simulink model "Off-Board-EV-Charger"  (R2018a)
settings: Solver=ode23tb  StartTime=0.0  StopTime=4  FixedStep=2.5e-6  MaxStep=1e-5  RelTol=1e-3  AbsTol=1e-5
undefined symbols (not defined in the file): Ion, Lithium
libraries: powerlib x22, simulink x7, powerlib_meascontrol x5, powerlib_extras x2, electricdrivelib x1, re_lib x1
settings Model: Creator=hp  LastModifiedBy=ADMIN
settings SolverCC: ZeroCrossControl=DisableAll  ZeroCrossAlgorithm=Adaptive  AlgebraicLoopSolver=LineSearch
settings DataIOCC: ReturnWorkspaceOutputs=on  Refine=2
settings DebuggingCC: AlgebraicLoopMsg=none  MaskedZcDiagnostic=none  IgnoredZcDiagnostic=none  UnconnectedInputMsg=none  UnconnectedOutputMsg=none  UnconnectedLineMsg=none
settings ModelReferenceCC: EnableRefExpFcnMdlSchedulingChecks=off
settings SFSimCC: SimUseLocalCustomCode=on
settings RTWCC: Description=Generic Real-Time Target  RTWUseLocalCustomCode=on

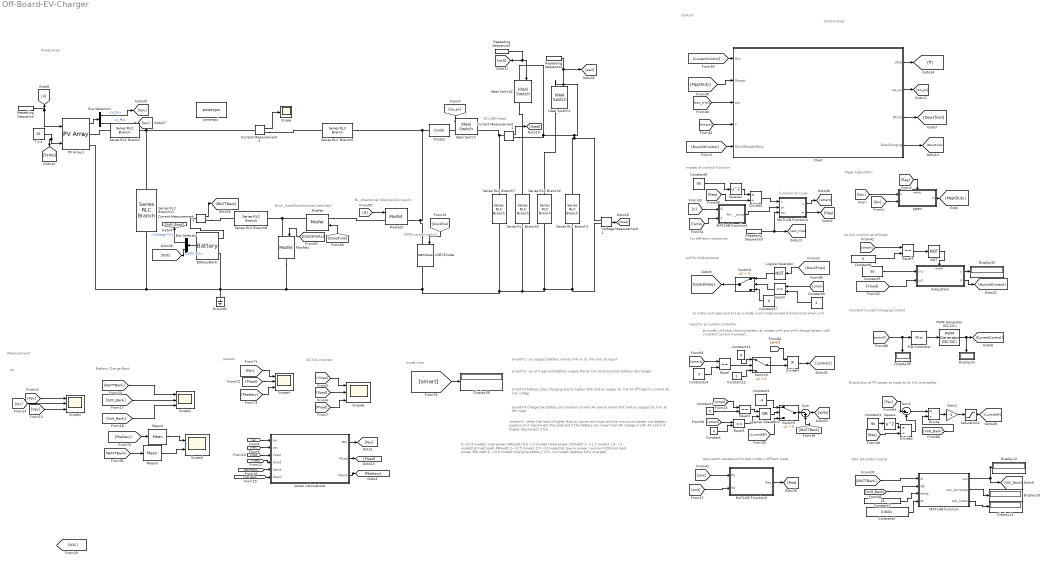
== system Off-Board-EV-Charger ==
  note: Buck_boost(bidrectional switches)
  note: DCLINK+load
  note: BI _directional (block/allow)
      | swich
  note: MPPt control switch
  note: mode view
  note: 0-->0.5 mode1( load power  306watt)
      | 0.5-->1 mode4 (load power  253watt)
      | 1-->1.5 mode3
      | 1.5-->2 mode2(at high load) 490watt
      | 2-->2.5 mode1
      | 2.5-->3 mode2(at low pv power ) pvmax=200 and load power 306 watt
      | 3-->3.5 mode5 (charging battery)
      | 3.5-->4 mode5 (battery fully charged
  note: dc link controll at offmppt
  note: Mppt Alghorithm
  note: Constant Current Charging Control
  note: powers
  note: DC link monitor
  note: Battery Charge Bank
  note: PV
  note: Measurement
  note: Control
  note: Power Area
  note: Distrbution of PV power at mppt to dc link and battey
  note: Control Area
  note: smart=1 : pv supplys battery and dc link or dc link only at mpp t
  note: smart=4 charge the battery at constant current 4A due to lower SOC and pv supplys dc link at off mppt
  note: smart=3 battery stop charging due to higher SOC and pv supply dc link at offmppt to control dc link voltge
  note: smart=5 : when the load is higher than pv power at mmpt and the maximum power can battery supplys so it disconnect the load and if the battery soc lower than 90 charge it with 4A and if it higher disconnect it too
  note: smart=2 : pv at mppt and battery supply the dc link (bidirectional battery discharge)
  note: function of mods
  note: for diffrent Irradiances
  note: modes of controll function
  note: sw3 for bidirectional
  note: to make sw3 open and act as a diode in all mods except bidirectional when y=2
  note: input for pi current controller
  note: at mode y=3 stop charing battery at modes y=5 and y=4 charge battery with constant current 4 ampers
  note: equivalent resistance for test mods in diffrent loads
  note: SOC Estimatorl trailer
  BatteryBank : electricdrivelib/Extra Sources/Battery  BatType=Lithium-Ion  ShowTempParam=off  ThermalPreset=no  ShowAgeParam=off  NomV=21.8  NomQ=12  SOC=80  Batt_Tr=1  PresetModel=on  MaxQ=12  MinV=16.35  FullV=25.3749  Dis_rate=5.2174  R=0.018167  Normal_OP=10.8522  expZone="[23.5524     0.589565]"  current=[6.5 13 32.5]  Units=Time  Tci=20  NomT=20  T2=-30  MaxQ2=4.8  FullV2=7.1  Normal_OP2=5.655  expZone2="[6.58           1]"  Rca=0.6  ti=2000  Dp=0  Neq0=0  Tsim=1e6  Ta1=25  Qeol=5.4*0.9  Reol=0.013333*1.2  Char_age=[2.3478, 3]  Dis_age=[2.3478, 10]  N1=1500  N2=10500  N3=1000  N4=1400  Ta2=45  N5=950
  Bus Selector : BusSelector  OutputSignals=Voltage (V),SOC (%)
  Bus Selector1 : BusSelector  OutputSignals=V_PV,I_PV
  Chart : Stateflow chart  TreatAsAtomicUnit=on
  Constant : Constant  Value=4
  Constant1 : Constant  Value=90
  Constant11 : Constant  Value=0
  Constant12 : Constant
  Constant17 : Constant  Value=0
  Constant2 : Constant  Value=0.0001
  Constant24 : Constant  Value=3
  Constant3 : Constant  Value=5
  Constant4 : Constant  Value=-4
  Constant5 : Constant  Value=90
  Constant6 : Constant  Value=5
  Constant7 : Constant  Value=25
  Constant8 : Constant  Value=2
  Constant9 : Constant  Value=90
  Current Measurement1 : powerlib/Measurements/Current Measurement  PhasorSimulation=off  OutputType=Complex  PSBequivalent=0
  Current Measurement2 : powerlib/Measurements/Current Measurement  PhasorSimulation=off  OutputType=Complex  PSBequivalent=0
  Current Measurement3 : powerlib/Measurements/Current Measurement  PhasorSimulation=off  OutputType=Complex  PSBequivalent=0
  Diode1 : powerlib/Power Electronics/Diode  Ron=0.001  Lon=0  Vf=0.8  IC=0  UseSnubber=0  Rs=500  Cs=250e-9  Measurements=off
  Display{10..12,30..31,33,38} (7 alike) : Display
  Divide : Product  Inputs=*/
  Divide2 : Product  Inputs=*/
  Divide4 : Product  Inputs=**
  Divide5 : Product  Inputs=*/
  Equal{,1..4} (5 alike) : RelationalOperator  Operator===  OutDataTypeStr=boolean  RndMeth=Simplest
  Gain1 : Gain  Gain=-1
  Ground2 : powerlib/Elements/Ground  LConnTagsString=a
  IGBT/Diode : powerlib/Power Electronics/IGBT//Diode  Ron=1e-3  Rs=1e5  Cs=inf  Measurements=on
  Ideal Switch : powerlib/Power Electronics/Ideal Switch  Ron=0.001  Lon=0  IC=0  Rs=1e5  Cs=inf  Measurements=on
  Ideal Switch1 : powerlib/Power Electronics/Ideal Switch  Ron=0.001  Lon=0  IC=0  Rs=1e5  Cs=inf  Measurements=on
  Ideal Switch2 : powerlib/Power Electronics/Ideal Switch  Ron=0.001  Lon=0  IC=0  Rs=1e5  Cs=inf  Measurements=on
  Logical Operator : Logic  Operator=NOT  AllPortsSameDT=off  OutDataTypeStr=boolean
  Logical Operator1 : Logic  Operator=OR  AllPortsSameDT=off  OutDataTypeStr=boolean
  MATLAB Function : MATLAB Function  TreatAsAtomicUnit=on
  MATLAB Function1 : MATLAB Function  TreatAsAtomicUnit=on
  MATLAB Function2 : MATLAB Function  TreatAsAtomicUnit=on
  MATLAB Function3 : MATLAB Function  TreatAsAtomicUnit=on
  MPPT : Subsystem
  Mean3 : powerlib_meascontrol/Measurements/Mean  Freq=50  Vinit=0  Ts=0
  Mean4 : powerlib_meascontrol/Measurements/Mean  Freq=50  Vinit=0  Ts=0
  Mosfet : powerlib/Power Electronics/Mosfet  Ron=0.1  Lon=0  Rd=0.01  Vfd=0  IC=0  Rs=1e5  Cs=inf  Measurements=on
  Mosfet1 : powerlib/Power Electronics/Mosfet  Ron=0.1  Lon=0  Rd=0.01  Vfd=0  IC=0  Rs=1e5  Cs=inf  Measurements=off
  Mosfet2 : powerlib/Power Electronics/Mosfet  Ron=0.1  Lon=0  Rd=0.01  Vfd=0  IC=0  Rs=1e5  Cs=inf  Measurements=on
  NOT : Logic  Operator=NOT  IconShape=distinctive  AllPortsSameDT=off  OutDataTypeStr=boolean
  PID Controller : simulink/Continuous/PID Controller  Controller=PI  TimeDomain=Continuous-time  SampleTime=-1  IntegratorMethod=Forward Euler  FilterMethod=Forward Euler  Form=Parallel  UseFilter=on  ControllerParametersSource=internal  P=25  I=5000  D=0  N=100  InitialConditionSource=internal  InitialConditionForIntegrator=0  InitialConditionForFilter=0  ExternalReset=none  LimitOutput=on  UpperSaturationLimit=0.95  LowerSaturationLimit=0  LinearizeAsGain=on  AntiWindupMode=clamping  Kb=1  TrackingMode=off  Kt=1  PParamMin=[]  PParamMax=[]  IParamMin=[]  IParamMax=[]  DParamMin=[]  DParamMax=[]  NParamMin=[]  NParamMax=[]  KbParamMin=[]  KbParamMax=[]  KtParamMin=[]  KtParamMax=[]  POutMin=[]  POutMax=[]  IOutMin=[]  IOutMax=[]  DOutMin=[]  DOutMax=[]  NOutMin=[]  NOutMax=[]  KbOutMin=[]  KbOutMax=[]  KtOutMin=[]  KtOutMax=[]  IntegratorOutMin=[]  IntegratorOutMax=[]  FilterOutMin=[]  FilterOutMax=[]  SumOutMin=[]  SumOutMax=[]  SumI1OutMin=[]  SumI1OutMax=[]  SumI2OutMin=[]  SumI2OutMax=[]  SumI3OutMin=[]  SumI3OutMax=[]  SumDOutMin=[]  SumDOutMax=[]  SaturationOutMin=[]  SaturationOutMax=[]  IntegratorContinuousStateAttributes=''  IntegratorStateMustResolveToSignalObject=off  IntegratorRTWStateStorageClass=Auto  FilterContinuousStateAttributes=''  FilterStateMustResolveToSignalObject=off  FilterRTWStateStorageClass=Auto  DifferentiatorICPrevScaledInput=0  DifferentiatorOutMin=[]  DifferentiatorOutMax=[]  FilterDiffOutCoefMin=[]  FilterDiffOutCoefMax=[]  SumDenOutMin=[]  SumDenOutMax=[]  SumNumOutMin=[]  SumNumOutMax=[]  ReciprocalOutMin=[]  ReciprocalOutMax=[]  DivideOutMin=[]  DivideOutMax=[]  TunerSelectOption=Transfer Function Based (PID Tuner App)
  PV Array1 : re_lib/Solar/PV Array  Npar=1  Nser=4  PlotType=array @ 25 deg.C & specified irradiances  S_vec="[ 1000   ]"  Temp_C_vec="[ 45 25  ]"  ModuleName=User-defined  PlotWhenSelected=off  Pm=99.925  Ncell=60  Voc=21.9  Isc=6.09  Vm=17.5  Im=5.71  beta_Voc_pc=-0.36099  alpha_Isc_pc=0.102  beta_Voc=-0.079057  alpha_Isc=0.0062118  IL=6.1019  I0=2.2502e-10  nI=0.59168  Rsh=284.8348  Rs=0.30531  BAL=off  Tc=1e-6  Tfilter=5e-5
  PWM Generator (DC-DC) : powerlib_meascontrol/Pulse & Signal Generators/PWM Generator (DC-DC)  Fsw=20000  Ts=0
  Repeating Sequence : simulink/Sources/Repeating Sequence  rep_seq_t="[0 2.5 2.5+1e-9 3  3.00000001 3.5 4]"  rep_seq_y="[1000 1000  500 500 250 250 250]"
  Repeating Sequence1 : simulink/Sources/Repeating Sequence  rep_seq_t=[0 0.5 0.5+1e-9 1.5 1.5+1e-9 4]  rep_seq_y=[1 1 0 0 1 1]
  Repeating Sequence2 : simulink/Sources/Repeating Sequence  rep_seq_t=[0 0.5 0.5+1e-9 1.5 1.5+1e-9 2 2.0000001 3.5 4]  rep_seq_y=[0 0 0 0 1 1 0 0 0]
  Repeating Sequence3 : simulink/Sources/Repeating Sequence  rep_seq_t=[0 0.5 1 1.5 2 2.5 3 3.5 4]  rep_seq_y=[10 50 90 90 50 70 10 90 90]
  Saturation2 : Saturate  UpperLimit=5  LowerLimit=-5
  Scope : Scope
  Scope{1..2,4,6} (4 alike) : Scope  NumInputPorts=3
  Scope3 : Scope  NumInputPorts=2
  Series RLC Branch : powerlib/Elements/Series RLC Branch  LConnTagsString=__new0  RConnTagsString=__new0  BranchType=R  Resistance=0.1  Inductance=1e-3  SetiL0=off  InitialCurrent=0  Capacitance=1e-6  Setx0=off  InitialVoltage=0  Measurements=None
  Series RLC Branch1 : powerlib/Elements/Series RLC Branch  LConnTagsString=__new0  RConnTagsString=__new0  BranchType=R  Resistance=32  Inductance=1e-3  SetiL0=off  InitialCurrent=0  Capacitance=0.0134  Setx0=off  InitialVoltage=50  Measurements=None
  Series RLC Branch11 : powerlib/Elements/Series RLC Branch  LConnTagsString=__new0  RConnTagsString=__new0  BranchType=C  Resistance=0.1  Inductance=1e-3  SetiL0=off  InitialCurrent=0  Capacitance=1000e-6  Setx0=off  InitialVoltage=0  Measurements=None
  Series RLC Branch2 : powerlib/Elements/Series RLC Branch  LConnTagsString=__new0  RConnTagsString=__new0  BranchType=R  Resistance=152.5  Inductance=1e-3  SetiL0=off  InitialCurrent=0  Capacitance=0.0134  Setx0=off  InitialVoltage=50  Measurements=None
  Series RLC Branch3 : powerlib/Elements/Series RLC Branch  LConnTagsString=__new0  RConnTagsString=__new0  BranchType=R  Resistance=43.86  Inductance=1e-3  SetiL0=off  InitialCurrent=0  Capacitance=0.0134  Setx0=off  InitialVoltage=50  Measurements=None
  Series RLC Branch6 : powerlib/Elements/Series RLC Branch  LConnTagsString=__new0  RConnTagsString=__new0  BranchType=L  Resistance=1  Inductance=13.5e-3  SetiL0=off  InitialCurrent=55  Capacitance=1e-6  Setx0=off  InitialVoltage=0  Measurements=None
  Series RLC Branch7 : powerlib/Elements/Series RLC Branch  LConnTagsString=__new0  RConnTagsString=__new0  BranchType=C  Resistance=0.0016  Inductance=1e-3  SetiL0=off  InitialCurrent=0  Capacitance=1000e-6  Setx0=off  InitialVoltage=50  Measurements=None
  Series RLC Branch8 : powerlib/Elements/Series RLC Branch  LConnTagsString=__new0  RConnTagsString=__new0  BranchType=L  Resistance=1  Inductance=3.5e-3  SetiL0=off  InitialCurrent=4  Capacitance=1e-6  Setx0=off  InitialVoltage=0  Measurements=None
  Square : Math  Operator=square  SaturateOnIntegerOverflow=on
  Square1 : Math  Operator=square  SaturateOnIntegerOverflow=on
  Subsystem : Subsystem
  Sum : Sum  Inputs=|-+
  Sum1 : Sum  Inputs=|+-
  Switch3 : Switch  Criteria=u2 > Threshold
  Switch4 : Switch  Criteria=u2 > Threshold
  Switch5 : Switch  Criteria=u2 > Threshold
  T in1 : Constant  Value=25
  Voltage Measurement1 : powerlib/Measurements/Voltage Measurement  PhasorSimulation=off  OutputType=Complex  PSBequivalent=0
  "power calculations " : Subsystem
  powergui : powerlib/powergui  Priority=1  SimulationMode=Discrete  SampleTime=5e-6  frequency=60  Iterations=50  frequencyindice=0  Pbase=100e6  ErrMax=1e-4  UnitsV=kV  UnitsW=MW  buscounter=0  FunctionMessages=off  echomessages=off  EnableUseOfTLC=off  CurrentSourceSwitches=off  DisableSnubberDevices=off  DisableRonSwitches=off  DisableVfSwitches=off  DisplayEquations=off  SolverType=Tustin/Backward Euler (TBE)  Interpol=off  ExternalGateDelay=off  methode=off  Ts=100  x0status=blocks  SPID=on  SwTol=0  HookPort=off  RestoreLinks=warning  ResistiveCurrentMeasurement=off  Frange=[0:2:500]  Ylog=off  Xlog=on  ShowGrid=off  save=off  variable=ZData  structure=0  ZoomFFT=off  StartTime=0.0  cycles=1  DisplayStyle=1  fundamental=60  FreqAxis=off  MaxFrequency=1000  frequencyindicesteady=1  RmsSteady=1  display=off
  wires:
  Current Measurement1/1 -> [Iload]
  T in1/1 -> PV Array1/2, [Temp]
  Bus Selector1/2 -> [Ipv]  "<I_PV>"
  Bus Selector1/1 -> [Vpv]  "<V_PV>"
  PV Array1/1 -> Bus Selector1/1
  Current Measurement3/1 -> [IBATTBank]
  BatteryBank/1 -> Bus Selector/1
  [Vload] -> Scope6/1
  [Iload] -> Scope6/2
  [Pload] -> Scope6/3
  [Ppv] -> Scope2/1
  Bus Selector/1 -> [Volt_Bank]  "<Voltage (V)>"
  [IBATTBank] -> Scope1/1
  [Volt_Bank] -> Scope1/3
  [SOC_Bank] -> Scope1/2
  PWM Generator (DC-DC)/1 -> [CurrentControl], Display31/1
  PID Controller/1 -> PWM Generator (DC-DC)/1
  [Ipv] -> MPPT/2(I)
  [Vpv] -> MPPT/1(V)
  Voltage Measurement1/1 -> [Vload]
  Divide/1 -> Gain1/1
  Sum1/1 -> Divide/1
  [Volt_Bank] -> Divide/2
  Bus Selector/2 -> [SOC]  "<SOC (%)>"
  [IBATTBank] -> Mean3/1
  Mean3/1 -> Scope3/2
  [BusVoltControl] -> Chart/5(DcLinkSupplyDuty)
  [CurrentControl] -> Chart/1(Dcc)
  Chart/3(Dfinal) -> [Dsw1final]
  Chart/4(DutyCharging) -> [Dsw2Final]
  Constant1/1 -> Square/1
  Square/1 -> Divide2/1
  Divide2/1 -> Sum1/2
  [control2] -> Display30/1, PID Controller/1
  [Dsw2Final] -> Mosfet/1
  Gain1/1 -> Saturation2/1
  Saturation2/1 -> [CurrentREF]
  [ff] -> Mosfet2/1
  [smart] -> Chart/4(Y)
  [DSW3FINAL] -> Mosfet1/1
  [MpptDuty] -> Chart/2(Dmppt)
  [Req] -> Divide2/2
  [Ppv] -> Sum1/1
  Chart/1(data) -> [ff]
  [Pbattery] -> Scope4/3
  [Ppv] -> Scope4/1
  [Pload] -> Scope4/2
  [smart] -> Display38/1
  MPPT/1(D) -> [MpptDuty]
  [flag] -> MPPT/Enable
  Chart/2(sw_pv) -> [sw_pv]
  [Dsw1final] -> IGBT/Diode/1
  [sw_pv] -> Ideal Switch/1
  [soc_trial] -> Chart/3(soc)
  Constant5/1 -> Subsystem/1(In1)
  [Vload] -> Subsystem/2(In2)
  Subsystem/1(y) -> Display33/1
  Subsystem/2(P) -> [BusVoltControl]
  NOT/1 -> Subsystem/Enable
  Equal4/1 -> NOT/1
  [smart] -> Equal4/1
  Constant6/1 -> Equal4/2
  Repeating Sequence/1 -> PV Array1/1, [Ir]
  Repeating Sequence1/1 -> Ideal Switch1/1, [sw2]
  Repeating Sequence2/1 -> [sw3], Ideal Switch2/1
  MATLAB Function2/1(y) -> [smart]
  Divide5/1 -> MATLAB Function2/1(u)
  MATLAB Function2/2(m) -> [flag]
  Square1/1 -> Divide5/1
  Constant9/1 -> Square1/1
  MATLAB Function1/1(Pmax_array) -> MATLAB Function2/2(pv)
  [Ir] -> MATLAB Function1/1(G)
  [Req] -> Divide5/2
  Repeating Sequence3/1 -> MATLAB Function2/3(soc), [soc_trial]
  [Temp] -> MATLAB Function1/2(T)
  Logical Operator/1 -> Switch4/1
  Constant17/1 -> Switch4/3
  [smart] -> Equal2/1
  [Dsw2Final] -> Logical Operator/1
  Constant8/1 -> Equal2/2
  Switch4/1 -> [DSW3FINAL]
  Equal2/1 -> Switch4/2
  Constant24/1 -> Equal/2
  Constant11/1 -> Switch3/1
  Equal3/1 -> Logical Operator1/1
  Logical Operator1/1 -> Switch5/2
  Switch5/1 -> Sum/1
  [smart] -> Equal1/1
  [diff2] -> Divide4/1
  [smart] -> Equal3/1
  Constant3/1 -> Equal3/2
  [CurrentREF] -> Switch5/3
  Constant/1 -> Equal1/2
  [IBATTBank] -> Sum/2
  Sum/1 -> [diff2]
  Equal/1 -> Switch3/2
  Divide4/1 -> [control2]
  Constant4/1 -> Switch5/1
  Equal1/1 -> Logical Operator1/2
  Switch3/1 -> Divide4/2
  [smart] -> Equal/1
  Constant12/1 -> Switch3/3
  [sw2] -> MATLAB Function3/1(R2)
  [sw3] -> MATLAB Function3/2(R3)
  MATLAB Function3/1(Req) -> [Req]
  [Pbattery] -> Mean4/1
  Mean4/1 -> Scope3/1
  [Ipv] -> "power calculations "/1("ipv ")
  [Vpv] -> "power calculations "/2("vpv ")
  "power calculations "/1("PPV ") -> [Ppv]
  "power calculations "/3(Pbank) -> [Pbattery]
  "power calculations "/2("Pload ") -> [Pload]
  [Iload] -> "power calculations "/3("iload ")
  [Vload] -> "power calculations "/4("vload ")
  [Volt_Bank] -> "power calculations "/6("vbank ")
  [IBATTBank] -> "power calculations "/5("ibank ")
  [Volt_Bank] -> MATLAB Function/2(VB)
  MATLAB Function/2(soc_corrected) -> Display10/1
  [IBATTBank] -> MATLAB Function/1(Ib)
  Constant2/1 -> MATLAB Function/4(dt)
  MATLAB Function/1(soc) -> [SOC_Bank], Display12/1
  Constant7/1 -> MATLAB Function/3(temp)
  MATLAB Function/3(soc_status) -> Display11/1
  [Ipv] -> Scope2/2
  [Vpv] -> Scope2/3
  Current Measurement2/1 -> Scope/1
  connections:
  Ideal Switch/RConn1 -- Series RLC Branch7/LConn1 -- Current Measurement1/LConn1
  Current Measurement3/RConn1 -- Series RLC Branch8/LConn1
  Series RLC Branch8/RConn1 -- Mosfet1/LConn1 -- Mosfet/RConn1
  Current Measurement1/RConn1 -- Ideal Switch2/LConn1 -- Ideal Switch1/LConn1 -- Series RLC Branch1/LConn1 -- Voltage Measurement1/LConn1
  IGBT/Diode/LConn1 -- Mosfet2/RConn1 -- Series RLC Branch6/RConn1 -- Diode1/LConn1
  Current Measurement3/LConn1 -- BatteryBank/LConn1
  Mosfet/LConn1 -- Mosfet2/LConn1
  Ideal Switch1/RConn1 -- Series RLC Branch2/LConn1
  Ideal Switch2/RConn1 -- Series RLC Branch3/LConn1
  PV Array1/RConn1 -- Series RLC Branch/LConn1
  Series RLC Branch/RConn1 -- Series RLC Branch11/LConn1 -- Current Measurement2/LConn1
  Ideal Switch/LConn1 -- Diode1/RConn1
  IGBT/Diode/RConn1 -- Series RLC Branch7/RConn1 -- Voltage Measurement1/LConn2 -- Series RLC Branch1/RConn1 -- Series RLC Branch2/RConn1 -- Series RLC Branch3/RConn1 -- Mosfet1/RConn1 -- PV Array1/RConn2 -- Series RLC Branch11/RConn1 -- Ground2/LConn1 -- BatteryBank/LConn2
  Current Measurement2/RConn1 -- Series RLC Branch6/LConn1

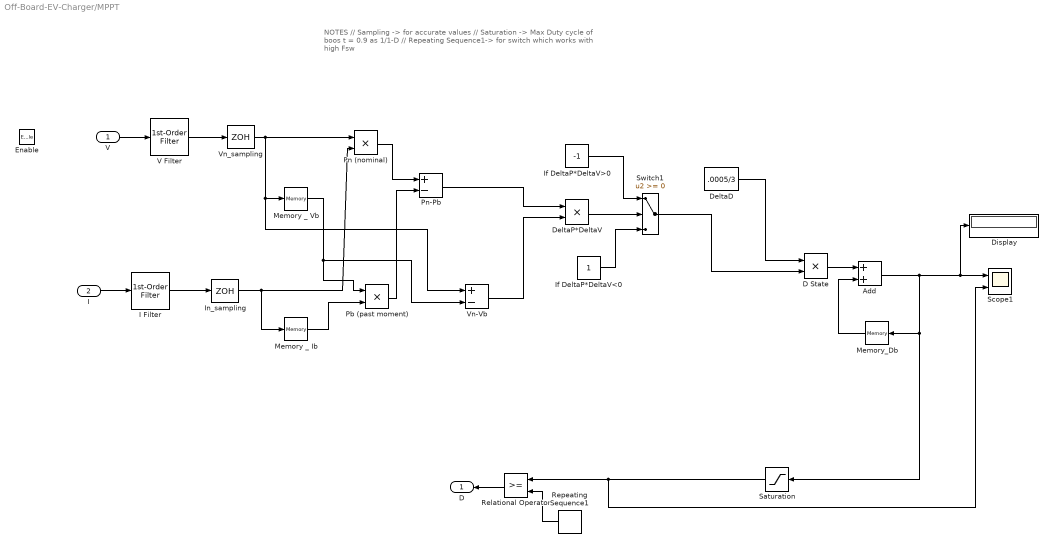
== system Off-Board-EV-Charger/MPPT ==
  note: NOTES
      | // Sampling -> for accurate values
      | // Saturation -> Max Duty cycle of boos t = 0.9 as 1/1-D
      | // Repeating Sequence1-> for switch which works with high Fsw
  V : Inport
  I : Inport  Port=2
  Enable : EnablePort
  Add : Sum
  D State : Product  RndMeth=Zero
  DeltaD : Constant  Value=.0005/3
  DeltaP*DeltaV : Product  RndMeth=Zero
  Display : Display
  I Filter : powerlib_extras/Control  Blocks/1st-Order  Filter  FilterType=Lowpass  Tc=1e-3  Initialize=off  Vac_Init=[0.8 -25 60]  Vdc_Init=-0.4  PlotResponse=off  param1=[1 500 1]
  If DeltaP*DeltaV<0 : Constant
  If DeltaP*DeltaV>0 : Constant  Value=-1
  "In_sampling " : ZeroOrderHold  SampleTime=1e-4
  Memory _ Ib : Memory  InheritSampleTime=on  LinearizeAsDelay=on
  Memory _ Vb : Memory  InheritSampleTime=on  LinearizeAsDelay=on
  Memory_Db : Memory  InheritSampleTime=on  LinearizeAsDelay=on
  Pb (past moment) : Product  RndMeth=Zero
  Pn (nominal) : Product  RndMeth=Zero
  Pn-Pb : Sum  Inputs=+-
  Relational Operator : RelationalOperator  OutDataTypeStr=boolean  RndMeth=Nearest
  Repeating Sequence1 : simulink/Sources/Repeating Sequence  rep_seq_t=[0 1/3000]  rep_seq_y=[0 1]
  Saturation : Saturate  UpperLimit=0.9  LowerLimit=0
  Scope1 : Scope  NumInputPorts=2
  Switch1 : Switch
  V Filter : powerlib_extras/Control  Blocks/1st-Order  Filter  FilterType=Lowpass  Tc=1e-3  Initialize=off  Vac_Init=[0.8 -25 60]  Vdc_Init=-0.4  PlotResponse=off  param1=[1 500 1]
  Vn-Vb : Sum  Inputs=+-
  Vn_sampling : ZeroOrderHold  SampleTime=1e-4
  D : Outport  VectorParamsAs1DForOutWhenUnconnected=on
  wires:
  V/1 -> V Filter/1
  I/1 -> I Filter/1
  V Filter/1 -> Vn_sampling/1
  I Filter/1 -> "In_sampling "/1
  "In_sampling "/1 -> Memory _ Ib/1, Pn (nominal)/2
  Vn_sampling/1 -> Pn (nominal)/1, Memory _ Vb/1, Vn-Vb/1
  Memory _ Ib/1 -> Pb (past moment)/2
  Memory _ Vb/1 -> Pb (past moment)/1, Vn-Vb/2
  Pn (nominal)/1 -> Pn-Pb/1
  Pb (past moment)/1 -> Pn-Pb/2
  D State/1 -> Add/1
  Repeating Sequence1/1 -> Relational Operator/2
  Relational Operator/1 -> D/1
  Memory_Db/1 -> Add/2
  Add/1 -> Saturation/1, Memory_Db/1, Display/1, Scope1/1
  Pn-Pb/1 -> DeltaP*DeltaV/1
  Vn-Vb/1 -> DeltaP*DeltaV/2
  DeltaP*DeltaV/1 -> Switch1/2
  If DeltaP*DeltaV>0/1 -> Switch1/1
  If DeltaP*DeltaV<0/1 -> Switch1/3
  DeltaD/1 -> D State/1
  Saturation/1 -> Relational Operator/1, Scope1/2
  Switch1/1 -> D State/2

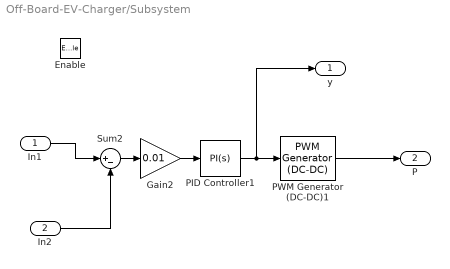
== system Off-Board-EV-Charger/Subsystem ==
  In1 : Inport
  In2 : Inport  Port=2
  Enable : EnablePort
  Gain2 : Gain  Gain=0.01
  PID Controller1 : simulink/Continuous/PID Controller  Controller=PI  TimeDomain=Continuous-time  SampleTime=-1  IntegratorMethod=Forward Euler  FilterMethod=Forward Euler  Form=Parallel  UseFilter=on  ControllerParametersSource=internal  P=0.8  I=5  D=1  N=100  InitialConditionSource=internal  InitialConditionForIntegrator=0  InitialConditionForFilter=0  ExternalReset=none  LimitOutput=on  UpperSaturationLimit=inf  LowerSaturationLimit=0  LinearizeAsGain=on  AntiWindupMode=clamping  Kb=1  TrackingMode=off  Kt=1  PParamMin=[]  PParamMax=[]  IParamMin=[]  IParamMax=[]  DParamMin=[]  DParamMax=[]  NParamMin=[]  NParamMax=[]  KbParamMin=[]  KbParamMax=[]  KtParamMin=[]  KtParamMax=[]  POutMin=[]  POutMax=[]  IOutMin=[]  IOutMax=[]  DOutMin=[]  DOutMax=[]  NOutMin=[]  NOutMax=[]  KbOutMin=[]  KbOutMax=[]  KtOutMin=[]  KtOutMax=[]  IntegratorOutMin=[]  IntegratorOutMax=[]  FilterOutMin=[]  FilterOutMax=[]  SumOutMin=[]  SumOutMax=[]  SumI1OutMin=[]  SumI1OutMax=[]  SumI2OutMin=[]  SumI2OutMax=[]  SumI3OutMin=[]  SumI3OutMax=[]  SumDOutMin=[]  SumDOutMax=[]  SaturationOutMin=[]  SaturationOutMax=[]  IntegratorContinuousStateAttributes=''  IntegratorStateMustResolveToSignalObject=off  IntegratorRTWStateStorageClass=Auto  FilterContinuousStateAttributes=''  FilterStateMustResolveToSignalObject=off  FilterRTWStateStorageClass=Auto  DifferentiatorICPrevScaledInput=0  DifferentiatorOutMin=[]  DifferentiatorOutMax=[]  FilterDiffOutCoefMin=[]  FilterDiffOutCoefMax=[]  SumDenOutMin=[]  SumDenOutMax=[]  SumNumOutMin=[]  SumNumOutMax=[]  ReciprocalOutMin=[]  ReciprocalOutMax=[]  DivideOutMin=[]  DivideOutMax=[]  TunerSelectOption=Transfer Function Based (PID Tuner App)
  PWM Generator (DC-DC)1 : powerlib_meascontrol/Pulse & Signal Generators/PWM Generator (DC-DC)  Fsw=3000  Ts=0
  Sum2 : Sum  Inputs=|+-
  y : Outport  VectorParamsAs1DForOutWhenUnconnected=on
  P : Outport  Port=2  VectorParamsAs1DForOutWhenUnconnected=on
  wires:
  PID Controller1/1 -> y/1, PWM Generator (DC-DC)1/1
  Sum2/1 -> Gain2/1
  Gain2/1 -> PID Controller1/1
  In2/1 -> Sum2/2
  In1/1 -> Sum2/1
  PWM Generator (DC-DC)1/1 -> P/1

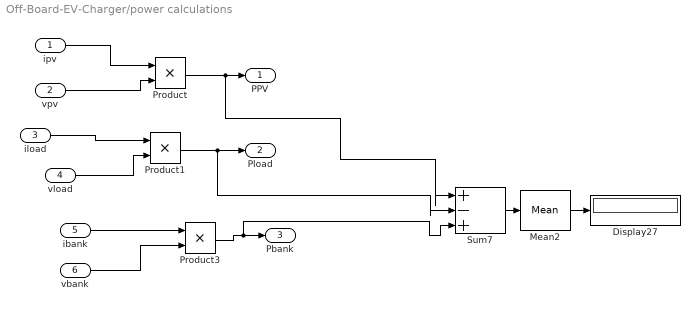
== system Off-Board-EV-Charger/power calculations  ==
  "ipv " : Inport
  "vpv " : Inport  Port=2
  "iload " : Inport  Port=3
  "vload " : Inport  Port=4
  "ibank " : Inport  Port=5
  "vbank " : Inport  Port=6
  Display27 : Display
  Mean2 : powerlib_meascontrol/Measurements/Mean  Freq=60  Vinit=0  Ts=0
  Product : Product
  Product1 : Product
  Product3 : Product
  Sum7 : Sum  Inputs=|+-+
  "PPV " : Outport
  "Pload " : Outport  Port=2
  Pbank : Outport  Port=3
  wires:
  "vload "/1 -> Product1/2
  "vpv "/1 -> Product/2
  Mean2/1 -> Display27/1
  "ibank "/1 -> Product3/1
  "iload "/1 -> Product1/1
  Product/1 -> Sum7/1, "PPV "/1
  Product1/1 -> Sum7/2, "Pload "/1
  Sum7/1 -> Mean2/1
  "vbank "/1 -> Product3/2
  Product3/1 -> Sum7/3, Pbank/1
  "ipv "/1 -> Product/1

== matlab function Off-Board-EV-Charger/MATLAB Function1 ==
  data: G input; T input; Pmax_array output
function Pmax_array  = fcn(G, T)
% ==================================================

P_STC     = 99.925;     % [W]      Maximum power at STC per module
Voc       = 21.9;       % [V]      Open circuit voltage
Isc       = 6.09;       % [A]      Short circuit current
Vmp       = 17.5;       % [V]      Voltage at MPP
Imp       = 5.71;       % [A]      Current at MPP

% Temperature coefficients from your block
alpha_Isc =  0.102;     % [%/°C]   Temp coeff of Isc
beta_Voc  = -0.36099;   % [%/°C]   Temp coeff of Voc

% ----------------------------------------------------------
%  ARRAY CONFIGURATION — from your Simulink block
% ----------------------------------------------------------
Ns = 4;    % series modules per string
Np = 1;    % parallel strings
N_modules  = Ns * Np;   % = 4 total modules

% ----------------------------------------------------------
%  POWER TEMPERATURE COEFFICIENT γ
%  Calculated from your module data — not assumed
%
%  γ = (alpha_Isc/100) + (beta_Voc/100)
%  This is the standard approximation for γ from datasheet
%  coefficients — matches the formula in your image
% ----------------------------------------------------------
gamma = (alpha_Isc / 100) + (beta_Voc / 100);
% gamma = (0.102/100) + (-0.36099/100) = -0.00259 /°C
% i.e. approximately -0.26%/°C — typical for silicon PV

% ----------------------------------------------------------
%  SAFETY CLAMPS — physical limits
% ----------------------------------------------------------
G = max(G, 0);          % irradiance cannot be negative
T = max(T, -40);        % temperature lower bound

% ----------------------------------------------------------
%  PMAX CALCULATION — single module
%  Pmax = P_STC × (G/1000) × [1 + γ×(T - 25)]
% ----------------------------------------------------------
Pmax = P_STC * (G / 1000) * (1 + gamma * (T - 25));
Pmax = max(Pmax, 0);    % power cannot be negative

% ----------------------------------------------------------
%  FULL ARRAY POWER
%  Series modules scale voltage, not power directly
%  but total array power = N_modules × single module power
% ----------------------------------------------------------
Pmax_array = N_modules * Pmax;

end

== matlab function Off-Board-EV-Charger/MATLAB Function ==
  settings: updateMethod=DISCRETE
  data: Ib input; soc output; VB input; temp input; soc_corrected output; dt input; soc_status output
function [soc, soc_corrected, soc_status] = fcn(Ib, VB, temp, dt)
% ==========================================================
%  SOC ESTIMATOR — 24V 12Ah 6S Li-ion Battery
%  Microohm Egypt | Built-in 6S BMS
% ==========================================================
%  INPUTS:
%   Ib   : Battery current [A]  (+ve = discharge, -ve = charge)
%   VB   : Battery terminal voltage [V]
%   temp : Battery temperature     [°C]
%   dt   : Sample time             [s]
%
%  OUTPUTS:
%   soc           : Coulomb-counted SOC     [%]
%   soc_corrected : OCV-corrected SOC       [%]
%   soc_status    : 0=OK 1=LOW 2=CRITICAL 3=FULL 4=OVERCHARGE 5=OVERDISCHARGE
% ==========================================================

persistent soc_p soc_corr_p

% ----------------------------------------------------------
%  PACK PARAMETERS — from datasheet
% ----------------------------------------------------------
Q_NOM          = 12;       % Nominal capacity            [Ah]
V_FULL         = 25.2;     % Fully charged voltage       [V]  4.2V × 6S
V_NOM          = 22.2;     % Nominal voltage             [V]  3.7V × 6S
V_CUTOFF       = 18.0;     % BMS under-voltage cutoff    [V]  3.0V × 6S
I_MAX_DIS      = 10.0;     % Max discharge current       [A]
I_MAX_CHG      = 5.0;      % Max charge current          [A]
ETA_CHARGE     = 0.98;     % Lithium charge efficiency
ETA_DISCHARGE  = 1.00;     % Discharge efficiency
SOC_INIT       = 50;       % Startup assumption          [%]

% ----------------------------------------------------------
%  SOC STATUS THRESHOLDS
% ----------------------------------------------------------
SOC_FULL       = 100;
SOC_HIGH       = 95;       % Approaching full
SOC_LOW        = 20;       % Low warning
SOC_CRITICAL   = 10;       % Critical — stop load

% ----------------------------------------------------------
%  INITIALISE PERSISTENTS
% ----------------------------------------------------------
if isempty(soc_p)
    soc_p      = SOC_INIT;
    soc_corr_p = SOC_INIT;
end

% ----------------------------------------------------------
%  TEMPERATURE DERATING
%  Li-ion loses ~0.5%/°C below 25°C, ~0.3%/°C above 45°C
% ----------------------------------------------------------
T_REF = 25;
if temp < T_REF
    k_temp = 0.005;                        % cold derating
else
    k_temp = 0.003;                        % heat derating
end
Q_eff = Q_NOM * (1 - k_temp * abs(temp - T_REF));
Q_eff = max(Q_eff, 0.5 * Q_NOM);          % floor at 50% of Q_NOM

% ----------------------------------------------------------
%  CURRENT CLAMPING — respect BMS limits
% ----------------------------------------------------------
Ib_safe = max(-I_MAX_CHG, min(I_MAX_DIS, Ib));

% ----------------------------------------------------------
%  COULOMB COUNTING
%  ΔSOC = (η × Ib × dt) / (Q_eff [As]) × 100
%  +Ib = discharging → SOC falls
%  -Ib = charging    → SOC rises
% ----------------------------------------------------------
if Ib_safe <= 0
    eta = ETA_CHARGE;
else
    eta = ETA_DISCHARGE;
end

delta_soc = (eta * Ib_safe * dt) / (Q_eff * 3600) * 100;
soc_new   = soc_p - delta_soc;
soc_new   = max(0, min(100, soc_new));
soc_p     = soc_new;

% ----------------------------------------------------------
%  OCV LOOKUP TABLE — 6S Li-ion pack (measured at rest)
%
%   Cell V :  3.00  3.30  3.50  3.60  3.65  3.70
%   Pack V :  18.0  19.8  21.0  21.6  21.9  22.2
%   SOC %  :     0    10    20    30    40    50
%
%   Cell V :  3.75  3.80  3.85  3.95  4.10  4.20
%   Pack V :  22.5  22.8  23.1  23.7  24.6  25.2
%   SOC %  :    60    70    80    90    95   100
% ----------------------------------------------------------
OCV_V   = [18.0, 19.8, 21.0, 21.6, 21.9, 22.2, ...
           22.5, 22.8, 23.1, 23.7, 24.6, 25.2];   % [V]
OCV_SOC = [  0,   10,   20,   30,   40,   50, ...
            60,   70,   80,   90,   95,  100];    % [%]

% Only correct when current is near zero (pack at equilibrium)
I_IDLE  = 1.0;     % [A] threshold for OCV to be valid
ALPHA   = 0.02;    % blend gain — smooth, no jumps

if abs(Ib) < I_IDLE && VB >= V_CUTOFF && VB <= V_FULL
    soc_ocv    = interp1(OCV_V, OCV_SOC, VB, 'linear', 'extrap');
    soc_ocv    = max(0, min(100, soc_ocv));
    soc_corr_p = soc_corr_p + ALPHA * (soc_ocv - soc_corr_p);
else
    % Track Coulomb counter while current flows
    soc_corr_p = soc_corr_p + ALPHA * (soc_p - soc_corr_p);
end

% ----------------------------------------------------------
%  STATUS FLAGS
% ----------------------------------------------------------
if VB > V_FULL
    soc_status = 4;          % OVERCHARGE — BMS should trigger
elseif VB < V_CUTOFF
    soc_status = 5;          % OVER-DISCHARGE — BMS should trigger
elseif soc_corr_p >= SOC_FULL
    soc_status = 3;          % FULL
elseif soc_corr_p <= SOC_CRITICAL
    soc_status = 2;          % CRITICAL  — cut load immediately
elseif soc_corr_p <= SOC_LOW
    soc_status = 1;          % LOW WARNING
else
    soc_status = 0;          % NORMAL OPERATION
end

% ----------------------------------------------------------
%  OUTPUTS
% ----------------------------------------------------------
soc           = soc_p;
soc_corrected = soc_corr_p;

end

== stateflow chart Off-Board-EV-Charger/Chart ==
  state OFFMPPT_WITH_BATTERY
    entry:
    Dfinal= DcLinkSupplyDuty;
    DutyCharging=Dcc
    sw_pv=1
    data =0;
    during:
    Dfinal=DcLinkSupplyDuty;
    DutyCharging=Dcc
    data=0;
    sw_pv=1
  state MPPT_WITH_WITHOUT_BATTERY
    Dfinal = double(Dmppt);
    DutyCharging=Dcc
    data =0;
    sw_pv=1
    during:
    Dfinal = double(Dmppt);
    DutyCharging=Dcc
    data = 0;
    sw_pv=1
    end
  state MPPT_bidirectional
    Dfinal = double(Dmppt);
    DutyCharging=0
    data =1;
    sw_pv=1
    during:
    Dfinal = double(Dmppt);
    data = 1;
    DutyCharging=Dcc
    sw_pv=1
    end
  state OFFMPPT_WITHOUT_BATTERY
    entry:
    data=0;
    Dfinal = DcLinkSupplyDuty
    DutyCharging=0
    sw_pv=1
    during:
    Dfinal = DcLinkSupplyDuty
    DutyCharging=0
    data=0;
    sw_pv=1
  state destroy
    data=0;
    Dfinal = 0
    sw_pv=0
    if soc<90
    DutyCharging=Dcc
    else
    DutyCharging=0
    end
    during:
    Dfinal = 0
    data=0;
    sw_pv=0
    if soc<90
    DutyCharging=Dcc
    else
    DutyCharging=0
    end
  MPPT_WITH_WITHOUT_BATTERY -> OFFMPPT_WITH_BATTERY [order 1] : [Y==4  ]
  (default) -> MPPT_WITH_WITHOUT_BATTERY
  OFFMPPT_WITH_BATTERY -> MPPT_WITH_WITHOUT_BATTERY [order 2] : [Y==1]
  OFFMPPT_WITH_BATTERY -> destroy [order 4] : [Y==5]
  MPPT_bidirectional -> MPPT_WITH_WITHOUT_BATTERY [order 1] : [Y==1]
  destroy -> OFFMPPT_WITH_BATTERY [order 4] : [Y==4]
  OFFMPPT_WITH_BATTERY -> OFFMPPT_WITHOUT_BATTERY [order 1] : [Y==3]
  OFFMPPT_WITHOUT_BATTERY -> OFFMPPT_WITH_BATTERY [order 1] : [Y==4]
  OFFMPPT_WITH_BATTERY -> MPPT_bidirectional [order 3] : [Y==2]
  MPPT_bidirectional -> OFFMPPT_WITH_BATTERY [order 3] : [Y==4]
  destroy -> MPPT_WITH_WITHOUT_BATTERY [order 3] : [Y==1]
  MPPT_WITH_WITHOUT_BATTERY -> MPPT_bidirectional [order 3] : [Y==2]
  MPPT_WITH_WITHOUT_BATTERY -> destroy [order 4] : [Y==5]
  OFFMPPT_WITHOUT_BATTERY -> MPPT_WITH_WITHOUT_BATTERY [order 2] : [Y==1]
  MPPT_WITH_WITHOUT_BATTERY -> OFFMPPT_WITHOUT_BATTERY [order 2] : [ Y==3 ]
  MPPT_bidirectional -> OFFMPPT_WITHOUT_BATTERY [order 2] : [Y==3]
  OFFMPPT_WITHOUT_BATTERY -> MPPT_bidirectional [order 3] : [Y==2]
  destroy -> MPPT_bidirectional [order 2] : [Y==2]
  MPPT_bidirectional -> destroy [order 4] : [[Y==5]]
  OFFMPPT_WITHOUT_BATTERY -> destroy [order 4] : [Y==5]
  destroy -> OFFMPPT_WITHOUT_BATTERY [order 1] : [Y==3]
  data: data output; sw_pv output; Dcc input; Dmppt input; soc input; Dfinal output double; DutyCharging output double; Y input; DcLinkSupplyDuty input

== matlab function Off-Board-EV-Charger/MATLAB Function2 ==
  data: u input; pv input; soc input; y output; m output
function [y,m]= fcn(u,pv, soc)

if u >= pv-125 && u<=pv && soc<=85
    y = 1;
    m=true;

elseif u > pv && u<pv+130 && soc >=20
    y = 2;
    m=true;
elseif (u < pv) && (soc > 85)   % stop PI of the battery
    y = 3;
    m = false;

elseif (u < pv-125) && (soc < 85)
    y = 4;
    m=false;
elseif (u>pv+130) || (soc<20 && u>pv)
    y=5;
    m= false;

else
    y = 0;
    m=true;

end

end

== matlab function Off-Board-EV-Charger/MATLAB Function3 ==
  data: Req output; R2 input; R3 input
function Req = equivalent_resistance(R2, R3)

% Parallel equivalent resistance
Req = 1 / ((1/32) + (R2/152.5) + (R3/43.86));

end
